simulink model "DroneGuard_Sim"  (R2026a)
settings: Solver=ode3  StopTime=T_end  FixedStep=Ts
undefined symbols (not defined in the file): Accel_max, Alt_cmd, Alt_init, BattFault_Slope, Cap_Ah, Cd_forward, g_accel, k_drain_fault, k_eff_fault, k_R_fault, K_therm, k_thrust, Kd_alt, Ki_alt, Ki_spd, Kp_alt, Kp_spd, m_drone, MotorFault_Slope, R_int, SOC_init, Speed_init, T_ambient, tau_therm, Ts, Use_Dynamic_RTH, V_empty, V_full
libraries: simulink x2, slpidlib x2
settings Model: Creator=admin  LastModifiedBy=admin

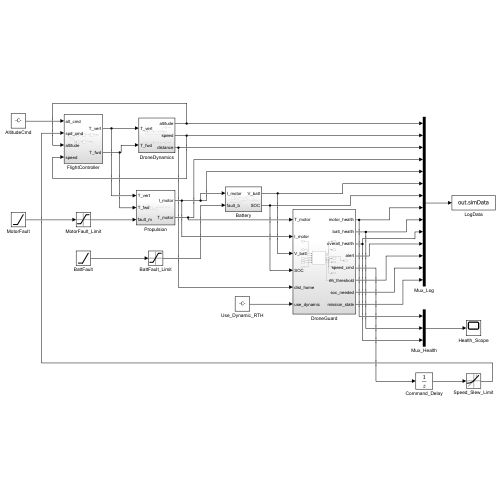
[thumbnail: Simulink's stored preview of the top-level diagram]
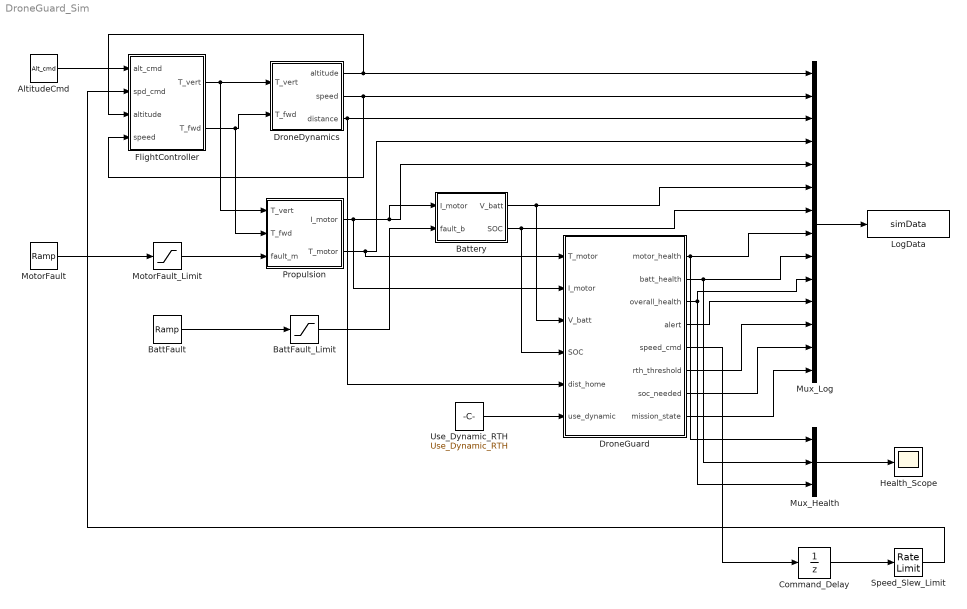
== system DroneGuard_Sim ==
  AltitudeCmd : Constant  Value=Alt_cmd
  BattFault : simulink/Sources/Ramp  slope=BattFault_Slope  start=BattFault_Start  InitialOutput=0
  BattFault_Limit : Saturate  UpperLimit=1  LowerLimit=0
  Battery : Subsystem
  Command_Delay : UnitDelay  SampleTime=Ts
  DroneDynamics : Subsystem
  DroneGuard : Subsystem
  FlightController : Subsystem
  Health_Scope : Scope
  LogData : ToWorkspace  VariableName=simData  SampleTime=-1
  MotorFault : simulink/Sources/Ramp  slope=MotorFault_Slope  start=MotorFault_Start  InitialOutput=0
  MotorFault_Limit : Saturate  UpperLimit=1  LowerLimit=0
  Mux_Health : Mux  Inputs=3
  Mux_Log : Mux  Inputs=14
  Propulsion : Subsystem
  Speed_Slew_Limit : RateLimiter  RisingSlewLimit=Accel_max  FallingSlewLimit=-Accel_max  SampleTimeMode=inherited
  Use_Dynamic_RTH : Constant  Value=Use_Dynamic_RTH
  wires:
  BattFault_Limit/1 -> Battery/2(fault_b)
  BattFault/1 -> BattFault_Limit/1
  MotorFault_Limit/1 -> Propulsion/3(fault_m)
  MotorFault/1 -> MotorFault_Limit/1
  DroneDynamics/1(altitude) -> Mux_Log/1, FlightController/3(altitude)
  DroneDynamics/2(speed) -> Mux_Log/2, FlightController/4(speed)
  FlightController/1(T_vert) -> Propulsion/1(T_vert), DroneDynamics/1(T_vert)
  FlightController/2(T_fwd) -> DroneDynamics/2(T_fwd), Propulsion/2(T_fwd)
  Propulsion/1(I_motor) -> Battery/1(I_motor), Mux_Log/5, DroneGuard/2(I_motor)
  Propulsion/2(T_motor) -> DroneGuard/1(T_motor), Mux_Log/4
  Battery/1(V_batt) -> Mux_Log/6, DroneGuard/3(V_batt)
  Battery/2(SOC) -> Mux_Log/7, DroneGuard/4(SOC)
  DroneDynamics/3(distance) -> DroneGuard/5(dist_home), Mux_Log/3
  DroneGuard/1(motor_health) -> Mux_Log/8, Mux_Health/1
  DroneGuard/2(batt_health) -> Mux_Log/9, Mux_Health/2
  DroneGuard/3(overall_health) -> Mux_Log/10, Mux_Health/3
  DroneGuard/4(alert) -> Mux_Log/11
  Mux_Log/1 -> LogData/1
  Speed_Slew_Limit/1 -> FlightController/2(spd_cmd)
  Use_Dynamic_RTH/1 -> DroneGuard/6(use_dynamic)
  DroneGuard/5(speed_cmd) -> Command_Delay/1
  Command_Delay/1 -> Speed_Slew_Limit/1
  DroneGuard/6(rth_threshold) -> Mux_Log/12
  DroneGuard/7(soc_needed) -> Mux_Log/13
  DroneGuard/8(mission_state) -> Mux_Log/14
  Mux_Health/1 -> Health_Scope/1
  AltitudeCmd/1 -> FlightController/1(alt_cmd)

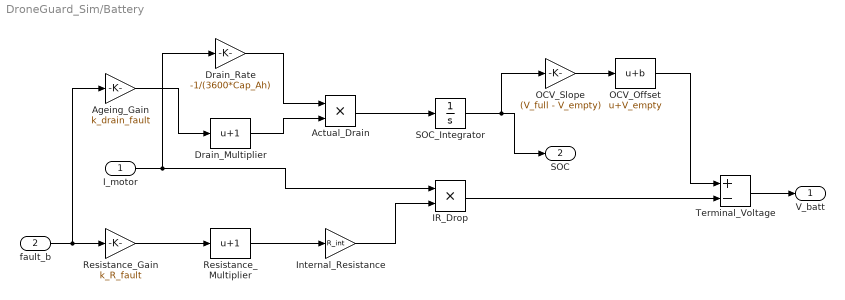
== system DroneGuard_Sim/Battery ==
  I_motor : Inport
  fault_b : Inport  Port=2
  Actual_Drain : Product
  Ageing_Gain : Gain  Gain=k_drain_fault
  Drain_Multiplier : Bias  Bias=1  SaturateOnIntegerOverflow=off
  Drain_Rate : Gain  Gain=-1/(3600*Cap_Ah)
  IR_Drop : Product
  Internal_Resistance : Gain  Gain=R_int
  OCV_Offset : Bias  Bias=V_empty  SaturateOnIntegerOverflow=off
  OCV_Slope : Gain  Gain=(V_full - V_empty)
  Resistance_Gain : Gain  Gain=k_R_fault
  Resistance_Multiplier : Bias  Bias=1  SaturateOnIntegerOverflow=off
  SOC_Integrator : Integrator  InitialCondition=SOC_init  LimitOutput=on  UpperSaturationLimit=1  LowerSaturationLimit=0
  Terminal_Voltage : Sum  Inputs=+-
  V_batt : Outport
  SOC : Outport  Port=2
  wires:
  Terminal_Voltage/1 -> V_batt/1
  IR_Drop/1 -> Terminal_Voltage/2
  OCV_Offset/1 -> Terminal_Voltage/1
  Internal_Resistance/1 -> IR_Drop/2
  Resistance_Multiplier/1 -> Internal_Resistance/1
  Resistance_Gain/1 -> Resistance_Multiplier/1
  OCV_Slope/1 -> OCV_Offset/1
  SOC_Integrator/1 -> OCV_Slope/1, SOC/1
  Actual_Drain/1 -> SOC_Integrator/1
  Drain_Multiplier/1 -> Actual_Drain/2
  Drain_Rate/1 -> Actual_Drain/1
  Ageing_Gain/1 -> Drain_Multiplier/1
  fault_b/1 -> Ageing_Gain/1, Resistance_Gain/1
  I_motor/1 -> Drain_Rate/1, IR_Drop/1

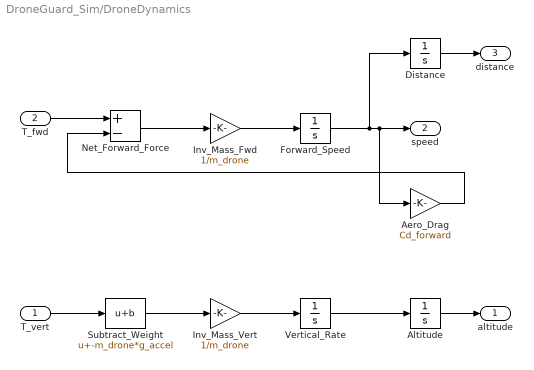
== system DroneGuard_Sim/DroneDynamics ==
  T_vert : Inport
  T_fwd : Inport  Port=2
  Aero_Drag : Gain  Gain=Cd_forward
  Altitude : Integrator  InitialCondition=Alt_init
  Distance : Integrator
  Forward_Speed : Integrator  InitialCondition=Speed_init
  Inv_Mass_Fwd : Gain  Gain=1/m_drone
  Inv_Mass_Vert : Gain  Gain=1/m_drone
  Net_Forward_Force : Sum  Inputs=+-
  Subtract_Weight : Bias  Bias=-m_drone*g_accel  SaturateOnIntegerOverflow=off
  Vertical_Rate : Integrator
  altitude : Outport
  speed : Outport  Port=2
  distance : Outport  Port=3
  wires:
  Distance/1 -> distance/1
  Aero_Drag/1 -> Net_Forward_Force/2
  Forward_Speed/1 -> speed/1, Aero_Drag/1, Distance/1
  Inv_Mass_Fwd/1 -> Forward_Speed/1
  Net_Forward_Force/1 -> Inv_Mass_Fwd/1
  T_fwd/1 -> Net_Forward_Force/1
  Altitude/1 -> altitude/1
  Vertical_Rate/1 -> Altitude/1
  Inv_Mass_Vert/1 -> Vertical_Rate/1
  Subtract_Weight/1 -> Inv_Mass_Vert/1
  T_vert/1 -> Subtract_Weight/1

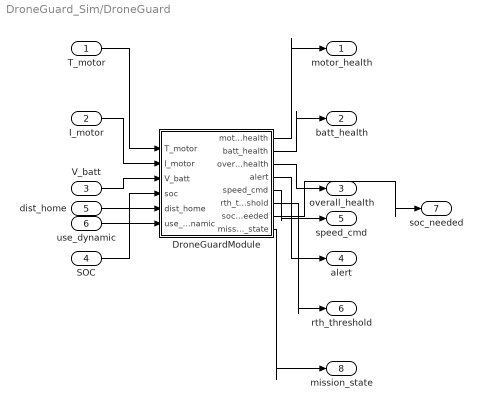
== system DroneGuard_Sim/DroneGuard ==
  T_motor : Inport
  I_motor : Inport  Port=2
  V_batt : Inport  Port=3
  SOC : Inport  Port=4
  dist_home : Inport  Port=5
  use_dynamic : Inport  Port=6
  DroneGuardModule : MATLAB Function  TreatAsAtomicUnit=on
  motor_health : Outport
  batt_health : Outport  Port=2
  overall_health : Outport  Port=3
  alert : Outport  Port=4
  speed_cmd : Outport  Port=5
  rth_threshold : Outport  Port=6
  soc_needed : Outport  Port=7
  mission_state : Outport  Port=8
  wires:
  DroneGuardModule/4(alert) -> alert/1
  DroneGuardModule/3(overall_health) -> overall_health/1
  DroneGuardModule/2(batt_health) -> batt_health/1
  DroneGuardModule/1(motor_health) -> motor_health/1
  SOC/1 -> DroneGuardModule/4(soc)
  V_batt/1 -> DroneGuardModule/3(V_batt)
  I_motor/1 -> DroneGuardModule/2(I_motor)
  T_motor/1 -> DroneGuardModule/1(T_motor)
  DroneGuardModule/8(mission_state) -> mission_state/1
  DroneGuardModule/7(soc_needed) -> soc_needed/1
  DroneGuardModule/6(rth_threshold) -> rth_threshold/1
  DroneGuardModule/5(speed_cmd) -> speed_cmd/1
  use_dynamic/1 -> DroneGuardModule/6(use_dynamic)
  dist_home/1 -> DroneGuardModule/5(dist_home)

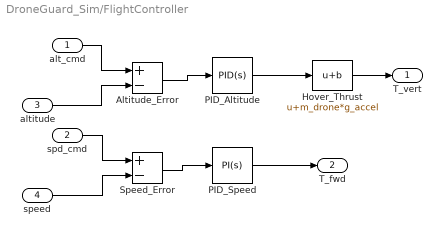
== system DroneGuard_Sim/FlightController ==
  alt_cmd : Inport
  spd_cmd : Inport  Port=2
  altitude : Inport  Port=3
  speed : Inport  Port=4
  Altitude_Error : Sum  Inputs=+-
  Hover_Thrust : Bias  Bias=m_drone*g_accel  SaturateOnIntegerOverflow=off
  PID_Altitude : slpidlib/PID Controller  Controller=PID  Form=Parallel  TimeDomain=Continuous-time  UseExternalTs=off  SampleTime=-1  IntegratorMethod=Forward Euler  FilterMethod=Forward Euler  ControllerParametersSource=internal  P=Kp_alt  I=Ki_alt  UseKiTs=off  D=Kd_alt  UseExternalDerivativeSource=off  N=100  UseFilter=on  TunerSelectOption=Transfer Function Based (PID Tuner App)  InitialConditionSource=internal  InitialConditionForIntegrator=0  InitialConditionForFilter=0  DifferentiatorICPrevScaledInput=0  ExternalReset=none  TrackingMode=off  Kt=1  LimitOutput=off  SatLimitsSource=internal  UpperSaturationLimit=inf  LowerSaturationLimit=-inf  LinearizeAsGain=on  AntiWindupMode=none  Kb=1  LimitIntegrator=off  UpperIntegratorSaturationLimit=inf  LowerIntegratorSaturationLimit=-inf  POutMin=[]  POutMax=[]  IOutMin=[]  IOutMax=[]  DOutMin=[]  DOutMax=[]  NOutMin=[]  NOutMax=[]  SumOutMin=[]  SumOutMax=[]  SaturationOutMin=[]  SaturationOutMax=[]  PParamMin=[]  PParamMax=[]  IParamMin=[]  IParamMax=[]  DParamMin=[]  DParamMax=[]  NParamMin=[]  NParamMax=[]  KbParamMin=[]  KbParamMax=[]  KtParamMin=[]  KtParamMax=[]  KbOutMin=[]  KbOutMax=[]  KtOutMin=[]  KtOutMax=[]  IntegratorOutMin=[]  IntegratorOutMax=[]  FilterOutMin=[]  FilterOutMax=[]  SumI1OutMin=[]  SumI1OutMax=[]  SumI2OutMin=[]  SumI2OutMax=[]  SumI3OutMin=[]  SumI3OutMax=[]  SumI4OutMin=[]  SumI4OutMax=[]  SumDOutMin=[]  SumDOutMax=[]  DifferentiatorOutMin=[]  DifferentiatorOutMax=[]  FilterDiffOutCoefMin=[]  FilterDiffOutCoefMax=[]  ReciprocalOutMin=[]  ReciprocalOutMax=[]  SumDenOutMin=[]  SumDenOutMax=[]  SumNumOutMin=[]  SumNumOutMax=[]  DivideOutMin=[]  DivideOutMax=[]  UdiffTsProdOutMin=[]  UdiffTsProdOutMax=[]  NTsProdOutMin=[]  NTsProdOutMax=[]  UintegralTsProdOutMin=[]  UintegralTsProdOutMax=[]  UngainTsProdOutMin=[]  UngainTsProdOutMax=[]  ClampingZeroOutDataTypeStr=Inherit: Inherit via back propagation  ClampingZeroOutMin=[]  ClampingZeroOutMax=[]  FilterDenConstantOutDataTypeStr=Inherit: Inherit via back propagation  FilterDenConstantOutMin=[]  FilterDenConstantOutMax=[]  PCopyOutDataTypeStr=Inherit: Inherit via back propagation  PCopyOutMin=[]  PCopyOutMax=[]  NCopyOutDataTypeStr=Inherit: Inherit via back propagation  NCopyOutMin=[]  NCopyOutMax=[]  IntegratorContinuousStateAttributes=''  IntegratorStateMustResolveToSignalObject=off  IntegratorRTWStateStorageClass=Auto  FilterContinuousStateAttributes=''  FilterStateMustResolveToSignalObject=off  FilterRTWStateStorageClass=Auto  ParallelPVariant=InternalParameters  IdealPVariant=Disabled  IVariant=InternalParameters  DVariant=InternalParameters  IntegratorVariant=Continuous  SatVariant=Disabled  AWVariant=Passthrough  PCopyVariant=Disabled  TRVariant=Disabled  FdbkBlocksVariant=Forward  IdealPFdbkVariant=Disabled  SatFdbkVariant=Disabled  DerivativeFilterVariant=ContFilter  NVariant=InternalParameters  NCopyVariant=Disabled  FilterICVariant=InternalICsFilter  IntegratorICVariant=InternalICs  ExternalResetVariant=Disabled  TRSumVariant=Passthrough  SumFdbkVariant=Disabled  SumVariant=Sum_PID  TsampFilterVariant=InternalTs  TsampNgainVariant=Passthrough  TsampIntegralVariant=Disabled_SignalSpec  ExternalSaturationOutDataTypeStr=Inherit: Same as second input  DerivativeSourceVariant=ErrorSignal  PreIntVariant=InternalPreInt
  PID_Speed : slpidlib/PID Controller  Controller=PI  Form=Parallel  TimeDomain=Continuous-time  UseExternalTs=off  SampleTime=-1  IntegratorMethod=Forward Euler  FilterMethod=Forward Euler  ControllerParametersSource=internal  P=Kp_spd  I=Ki_spd  UseKiTs=off  D=0  UseExternalDerivativeSource=off  N=100  UseFilter=on  TunerSelectOption=Transfer Function Based (PID Tuner App)  InitialConditionSource=internal  InitialConditionForIntegrator=Cd_forward*Speed_init  InitialConditionForFilter=0  DifferentiatorICPrevScaledInput=0  ExternalReset=none  TrackingMode=off  Kt=1  LimitOutput=off  SatLimitsSource=internal  UpperSaturationLimit=inf  LowerSaturationLimit=-inf  LinearizeAsGain=on  AntiWindupMode=none  Kb=1  LimitIntegrator=off  UpperIntegratorSaturationLimit=inf  LowerIntegratorSaturationLimit=-inf  POutMin=[]  POutMax=[]  IOutMin=[]  IOutMax=[]  DOutMin=[]  DOutMax=[]  NOutMin=[]  NOutMax=[]  SumOutMin=[]  SumOutMax=[]  SaturationOutMin=[]  SaturationOutMax=[]  PParamMin=[]  PParamMax=[]  IParamMin=[]  IParamMax=[]  DParamMin=[]  DParamMax=[]  NParamMin=[]  NParamMax=[]  KbParamMin=[]  KbParamMax=[]  KtParamMin=[]  KtParamMax=[]  KbOutMin=[]  KbOutMax=[]  KtOutMin=[]  KtOutMax=[]  IntegratorOutMin=[]  IntegratorOutMax=[]  FilterOutMin=[]  FilterOutMax=[]  SumI1OutMin=[]  SumI1OutMax=[]  SumI2OutMin=[]  SumI2OutMax=[]  SumI3OutMin=[]  SumI3OutMax=[]  SumI4OutMin=[]  SumI4OutMax=[]  SumDOutMin=[]  SumDOutMax=[]  DifferentiatorOutMin=[]  DifferentiatorOutMax=[]  FilterDiffOutCoefMin=[]  FilterDiffOutCoefMax=[]  ReciprocalOutMin=[]  ReciprocalOutMax=[]  SumDenOutMin=[]  SumDenOutMax=[]  SumNumOutMin=[]  SumNumOutMax=[]  DivideOutMin=[]  DivideOutMax=[]  UdiffTsProdOutMin=[]  UdiffTsProdOutMax=[]  NTsProdOutMin=[]  NTsProdOutMax=[]  UintegralTsProdOutMin=[]  UintegralTsProdOutMax=[]  UngainTsProdOutMin=[]  UngainTsProdOutMax=[]  ClampingZeroOutDataTypeStr=Inherit: Inherit via back propagation  ClampingZeroOutMin=[]  ClampingZeroOutMax=[]  FilterDenConstantOutDataTypeStr=Inherit: Inherit via back propagation  FilterDenConstantOutMin=[]  FilterDenConstantOutMax=[]  PCopyOutDataTypeStr=Inherit: Inherit via back propagation  PCopyOutMin=[]  PCopyOutMax=[]  NCopyOutDataTypeStr=Inherit: Inherit via back propagation  NCopyOutMin=[]  NCopyOutMax=[]  IntegratorContinuousStateAttributes=''  IntegratorStateMustResolveToSignalObject=off  IntegratorRTWStateStorageClass=Auto  FilterContinuousStateAttributes=''  FilterStateMustResolveToSignalObject=off  FilterRTWStateStorageClass=Auto  ParallelPVariant=InternalParameters  IdealPVariant=Disabled  IVariant=InternalParameters  DVariant=Disabled  IntegratorVariant=Continuous  SatVariant=Disabled  AWVariant=Passthrough  PCopyVariant=Disabled  TRVariant=Disabled  FdbkBlocksVariant=Forward  IdealPFdbkVariant=Disabled  SatFdbkVariant=Disabled  DerivativeFilterVariant=Disabled  NVariant=Disabled  NCopyVariant=Disabled_SignalSpec  FilterICVariant=Disabled  IntegratorICVariant=InternalICs  ExternalResetVariant=Disabled  TRSumVariant=Passthrough  SumFdbkVariant=Disabled  SumVariant=Sum_PI  TsampFilterVariant=InternalTs  TsampNgainVariant=Passthrough  TsampIntegralVariant=Disabled_SignalSpec  ExternalSaturationOutDataTypeStr=Inherit: Same as second input  DerivativeSourceVariant=Disabled  PreIntVariant=InternalPreInt
  Speed_Error : Sum  Inputs=+-
  T_vert : Outport
  T_fwd : Outport  Port=2
  wires:
  Hover_Thrust/1 -> T_vert/1
  speed/1 -> Speed_Error/2
  spd_cmd/1 -> Speed_Error/1
  altitude/1 -> Altitude_Error/2
  alt_cmd/1 -> Altitude_Error/1
  PID_Speed/1 -> T_fwd/1
  Speed_Error/1 -> PID_Speed/1
  PID_Altitude/1 -> Hover_Thrust/1
  Altitude_Error/1 -> PID_Altitude/1

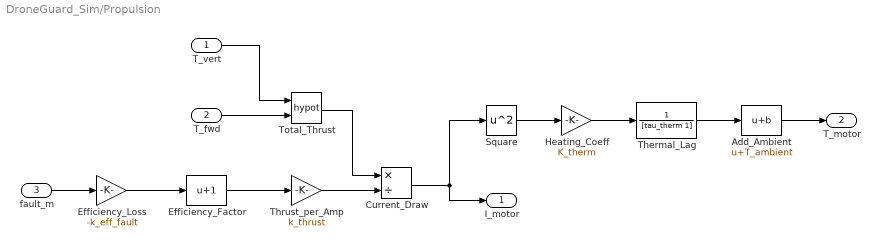
== system DroneGuard_Sim/Propulsion ==
  T_vert : Inport
  T_fwd : Inport  Port=2
  fault_m : Inport  Port=3
  Add_Ambient : Bias  Bias=T_ambient  SaturateOnIntegerOverflow=off
  Current_Draw : Product  Inputs=*/
  Efficiency_Factor : Bias  Bias=1  SaturateOnIntegerOverflow=off
  Efficiency_Loss : Gain  Gain=-k_eff_fault
  Heating_Coeff : Gain  Gain=K_therm
  Square : Math  Operator=square
  Thermal_Lag : TransferFcn  Denominator=[tau_therm 1]
  Thrust_per_Amp : Gain  Gain=k_thrust
  Total_Thrust : Math  Operator=hypot
  I_motor : Outport
  T_motor : Outport  Port=2
  wires:
  Add_Ambient/1 -> T_motor/1
  Thermal_Lag/1 -> Add_Ambient/1
  Heating_Coeff/1 -> Thermal_Lag/1
  Square/1 -> Heating_Coeff/1
  Current_Draw/1 -> I_motor/1, Square/1
  Thrust_per_Amp/1 -> Current_Draw/2
  Total_Thrust/1 -> Current_Draw/1
  Efficiency_Factor/1 -> Thrust_per_Amp/1
  Efficiency_Loss/1 -> Efficiency_Factor/1
  fault_m/1 -> Efficiency_Loss/1
  T_fwd/1 -> Total_Thrust/2
  T_vert/1 -> Total_Thrust/1

== matlab function DroneGuard_Sim/DroneGuard/DroneGuardModule ==
  settings: updateMethod=DISCRETE  sampleTime=Ts
  data: T_motor input; motor_health output; I_motor input; V_batt input; soc input; batt_health output; overall_health output; alert output; dist_home input; use_dynamic input; speed_cmd output; rth_threshold output; soc_needed output; mission_state output
function [motor_health, batt_health, overall_health, alert, speed_cmd, rth_threshold, soc_needed, mission_state] = DroneGuardModule(T_motor, I_motor, V_batt, soc, dist_home, use_dynamic)
%#codegen
% The entire DroneGuard companion computer - health scoring and mission
% optimisation as one loop, not two. The logic lives in droneguard_module.m
% so the identical code can be unit-tested in MATLAB and compiled for a Pi.
[motor_health, batt_health, overall_health, alert, speed_cmd, rth_threshold, soc_needed, mission_state] = ...
    droneguard_module(T_motor, I_motor, V_batt, soc, dist_home, use_dynamic);
end
